simulink model "case_19_all_state_oscillation"  (R2025b)
settings: Solver=VariableStepAuto  StartTime=0.0  StopTime=240  RelTol=1e-3
settings Model: Creator=sanborkl  LastModifiedBy=sanborkl

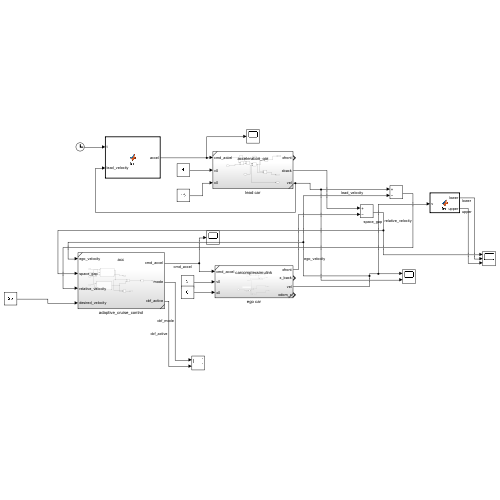
[thumbnail: Simulink's stored preview of the top-level diagram]
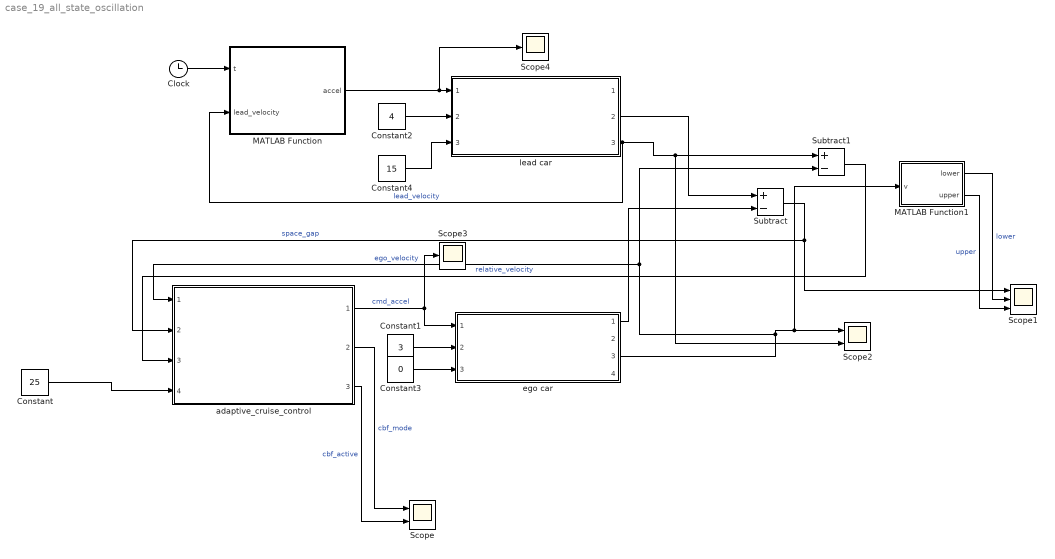
== system case_19_all_state_oscillation ==
  Clock : Clock
  Constant : Constant  Value=25
  Constant1 : Constant  Value=3
  Constant2 : Constant  Value=4
  Constant3 : Constant  Value=0
  Constant4 : Constant  Value=15
  MATLAB Function : MATLAB Function  TreatAsAtomicUnit=on
  MATLAB Function1 : MATLAB Function  TreatAsAtomicUnit=on
  Scope : Scope  NumInputPorts=2
      settings: ActiveDisplayYMinimum=0.75000000000000011  ActiveDisplayYMaximum=3.25
  Scope1 : Scope  NumInputPorts=3
      settings: ActiveDisplayYMinimum=1.9570427135336477  ActiveDisplayYMaximum=89.98661557819716  YLabel=m
  Scope2 : Scope  NumInputPorts=2
      settings: ActiveDisplayYMinimum=-1.6843921970909721  ActiveDisplayYMaximum=15.159529773818752  YLabel=m/s  DataLoggingVariableName=ScopeData2
  Scope3 : Scope
      settings: ActiveDisplayYMinimum=-1.9184197855824903  ActiveDisplayYMaximum=1.8798244206202765  YLabel=m/s^2  DataLoggingVariableName=ScopeData3
  Scope4 : Scope
      settings: ActiveDisplayYMinimum=-1.875  ActiveDisplayYMaximum=1.875  DataLoggingVariableName=ScopeData4
  Subtract : Sum  Inputs=+-
  Subtract1 : Sum  Inputs=+-
  adaptive_cruise_control : Subsystem  ReferencedSubsystem=acc
  ego car : Subsystem  ReferencedSubsystem=carcomplexsimulink
  lead car : Subsystem  ReferencedSubsystem=acceleration_car
  wires:
  ego car/3 -> Scope2/1, MATLAB Function1/1(v), Subtract1/2, adaptive_cruise_control/1  "ego_velocity"
  adaptive_cruise_control/1 -> ego car/1, Scope3/1  "cmd_accel"
  Constant1/1 -> ego car/2
  Subtract1/1 -> adaptive_cruise_control/3  "relative_velocity"
  lead car/3 -> MATLAB Function/2(lead_velocity), Scope2/2, Subtract1/1  "lead_velocity"
  Constant3/1 -> ego car/3
  Constant2/1 -> lead car/2
  adaptive_cruise_control/2 -> Scope/1  "cbf_mode"
  lead car/2 -> Subtract/1
  adaptive_cruise_control/3 -> Scope/2  "cbf_active"
  Constant/1 -> adaptive_cruise_control/4
  ego car/1 -> Subtract/2
  Subtract/1 -> Scope1/1, adaptive_cruise_control/2  "space_gap"
  Constant4/1 -> lead car/3
  MATLAB Function/1(accel) -> Scope4/1, lead car/1
  MATLAB Function1/1(lower) -> Scope1/2  "lower"
  MATLAB Function1/2(upper) -> Scope1/3  "upper"
  Clock/1 -> MATLAB Function/1(t)

== matlab function case_19_all_state_oscillation/MATLAB Function ==
  data: t input; accel output; lead_velocity input
function accel = fcn(t, lead_velocity)

cycle_time = 20;

t_adj = mod(floor(t), cycle_time);

if t_adj < cycle_time / 5.0
    if lead_velocity > (5.0 - 1)
        accel = -1.5;
        return
    end
else
    if lead_velocity < (7.5 + 1)
        accel = 1.5;
        return
    end
end

accel = 0;

== matlab function case_19_all_state_oscillation/MATLAB Function1 ==
  data: v input; lower output; upper output
function [lower, upper] = fcn(v)

lower = 2 * v + 5;
upper = 2 * v + 15;
